simulink subsystem "stab_pole_placement"  (R2026a)
settings: Solver=VariableStepAuto
undefined symbols (not defined in the file or in its folder): ctrlP
settings Model: Creator=ahmad  LastModifiedBy=ahmad

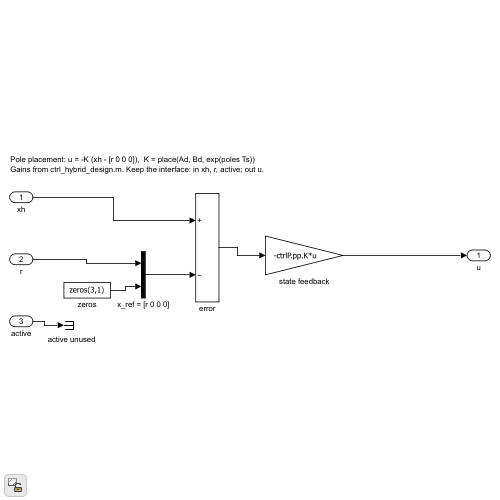
[thumbnail: Simulink's stored preview of the top-level diagram]
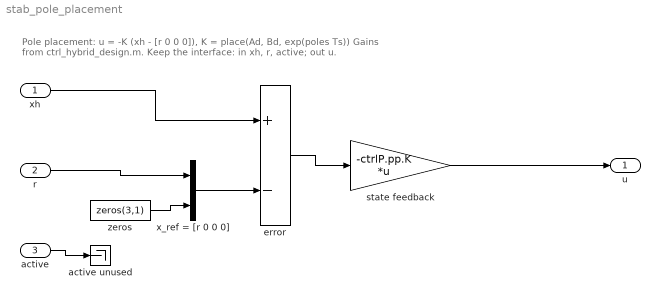
== system stab_pole_placement ==
  note: Pole placement: u = -K (xh - [r 0 0 0]),  K = place(Ad, Bd, exp(poles Ts))
      | Gains from ctrl_hybrid_design.m. Keep the interface: in xh, r, active; out u.
  xh : Inport  PortDimensions=4
  r : Inport  Port=2
  active : Inport  Port=3
  active unused : Terminator
  error : Sum  Inputs=+-
  state feedback : Gain  Gain=-ctrlP.pp.K  Multiplication=Matrix(K*u)
  x_ref = [r 0 0 0] : Mux  Inputs=[1 3]
  zeros : Constant  Value=zeros(3,1)
  u : Outport
  wires:
  r/1 -> x_ref = [r 0 0 0]/1
  zeros/1 -> x_ref = [r 0 0 0]/2
  xh/1 -> error/1
  x_ref = [r 0 0 0]/1 -> error/2
  error/1 -> state feedback/1
  state feedback/1 -> u/1
  active/1 -> active unused/1
